simulink model "walkingRobot"  (R2019a)
settings: Solver=ode15s  StartTime=0.0  StopTime=10  EnableMultiTasking=on
InitFcn:
  | initAnglesR = evalSmoothTrajectory(curveData,0);
  | initAnglesL = evalSmoothTrajectory(curveData,-curveData.gaitPeriod/2);
values from neighbouring files (symbols this model uses):
  ankle_servo_kd = 8    [robotParameters.m]
  ankle_servo_ki = 4    [robotParameters.m]
  ankle_servo_kp = 20    [robotParameters.m]
  curveData = createSmoothTrajectory(ankle_motion,knee_motion,hip_motion,gaitPeriod)    [robotParameters.m]
  deriv_filter_coeff = 100    [robotParameters.m]
  foot_x = 8    [robotParameters.m]
  foot_y = 6    [robotParameters.m]
  foot_z = 1    [robotParameters.m]
  height_plane = 0.025    [robotParameters.m]
  hip_servo_kd = 20    [robotParameters.m]
  hip_servo_ki = 10    [robotParameters.m]
  hip_servo_kp = 60    [robotParameters.m]
  joint_stiffness = 1    [robotParameters.m]
  knee_servo_kd = 10    [robotParameters.m]
  knee_servo_ki = 5    [robotParameters.m]
  knee_servo_kp = 60    [robotParameters.m]
  lower_leg_length = 10    [robotParameters.m]
  N = 500    [plotSmoothTrajectory.m]
  plane_x = 25    [robotParameters.m]
  plane_y = 3    [robotParameters.m]
  torso_offset_x = -0.5    [robotParameters.m]
  torso_offset_z = -2    [robotParameters.m]
  torso_x = 5    [robotParameters.m]
  torso_y = 10    [robotParameters.m]
  torso_z = 8    [robotParameters.m]
  upper_leg_length = 10    [robotParameters.m]
undefined symbols (not defined in the file or in its folder): X, Y, Z
libraries: sm_lib x29, walkingRobotUtils x12, Contact_Forces_Lib x8, nesl_utility x4, simulink x1
settings Model: Creator=scastro  LastModifiedBy=scastro
settings DataIOCC: ReturnWorkspaceOutputs=off  OutputTimes=0:0.01:10
settings OptimizationCC: LifeSpan=inf
settings DebuggingCC: AllowSymbolicDim=off  SFUnexpectedBacktrackingDiag=warning  SFNoUnconditionalDefaultTransitionDiag=warning  SFExecutionAtInitializationDiag=none  UnitsInconsistencyMsg=none  ArithmeticOperatorsInVariantConditions=warning
settings SFSimCC: SimUseLocalCustomCode=off
settings RTWCC: RTWUseLocalCustomCode=off
settings CodeAppCC: StateflowObjectComments=on
settings GRTTargetCC: TargetLangStandard=C89/C90 (ANSI)  GeneratePreprocessorConditionals=Disable all
settings ConfigComp: CovMetricSettings=dw  CovHtmlReporting=on  CovSaveCumulativeToWorkspaceVar=on  CovSaveSingleToWorkspaceVar=on  CovExternalEMLEnable=off  CovSFcnEnable=off
settings SimscapeCC: SimscapeNormalizeSystem=off  SimscapeLogOpenViewer=on  SimscapeLogLimitData=off  SimscapeLogDataHistory=10000
settings ConfigurationSet: Description=SimMechanics 2G
settings DiagnosticsConfigSet: SimMechanicsRigidlyBoundBlock=none
settings ExplorerConfigSet: InternalSimMechanicsExplorerSettings="<ExplorerConfiguration><canonicalview>default</canonicalview><AnimationSetting><BasePlaybackSpeed>1.0</BasePlaybackSpeed><PlaybackSpeedFactor>1.0</PlaybackSpeedFactor></AnimationSetting><TilePanel><TileInfo><Tiles Columns=\"1\" Count=\"1\" Rows=\"1\"><Column Left=\"2\" Weight=\"1\"/><Column Left=\"1242\"/><Row Top=\"2\" Weight=\"1\"/><Row Top=\"924\"/><Tile Height=\"1\" Width=\"1\" X=\"0\" Y=\"0\"/></Tiles></TileInfo><SceneInfo><SceneViewer><BGColor><R>0.60000002384185791</R><G>0.60000002384185791</G><B>0.60000002384185791</B></BGColor><Camera><DoPerspective>off</DoPerspective><Position><X>3.5288544276265377</X><Y>-3.5929715781454834</Y><Z>1.702213827013187</Z></Position><Center><X>1.5263892499290903</X><Y>0.59161729631936055</Y><Z>-0.28619491412557885</Z></Center><Up><X>-0.24511053110164599</X><Y>0.31791313039198377</Y><Z>0.91588867722416945</Z></Up><ViewLimDist>1</ViewLimDist><YLim>1.3675114445300658</YLim><XLim>1.8438188260859925</XLim></Camera></SceneViewer></SceneInfo></TilePanel><MechEditorPanel><Cameras/><GfxPanelCameraMap/><VideoCreator><PlaybackSpeedRatio>1.0</PlaybackSpeedRatio><FrameRate>30</FrameRate><VideoFormat>Motion JPEG AVI</VideoFormat><FrameSize>auto</FrameSize></VideoCreator></MechEditorPanel></ExplorerConfiguration>"

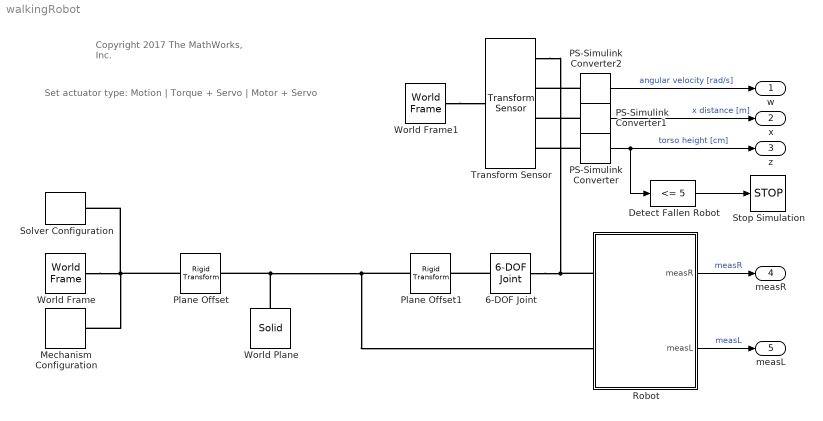
== system walkingRobot ==
  note: Set actuator type:
      | Motion | Torque + Servo | Motor + Servo
  note: Copyright 2017 The MathWorks, Inc.
  6-DOF Joint : sm_lib/Joints/6-DOF Joint  SenseConstraintForce=off  SenseConstraintForceX=off  SenseConstraintForceY=off  SenseConstraintForceZ=off  SenseConstraintTorque=off  SenseConstraintTorqueX=off  SenseConstraintTorqueY=off  SenseConstraintTorqueZ=off  SenseTotalForce=off  SenseTotalForceX=off  SenseTotalForceY=off  SenseTotalForceZ=off  SenseTotalTorque=off  SenseTotalTorqueX=off  SenseTotalTorqueY=off  SenseTotalTorqueZ=off  CompositeWrenchDir=FollowerOnBase  CompositeWrenchFrame=BaseFrame  PxEquilibriumPosition=0  PxEquilibriumPositionUnits=m  PxSpringStiffness=0  PxSpringStiffnessUnits=N/m  PxDampingCoefficient=world_damping  PxDampingCoefficientUnits=N/(m/s)  PxTorqueActuationMode=NoTorque  PxMotionActuationMode=ComputedMotion  PxSensePosition=off  PxSenseVelocity=off  PxSenseAcceleration=off  PxSenseTorqueForce=off  PxSenseLowerLimitTorqueForce=off  PxSenseUpperLimitTorqueForce=off  PxLowerLimitSpecify=off  PxLowerLimitBound=-1  PxLowerLimitBoundUnits=m  PxLowerLimitStiffness=1e6  PxLowerLimitStiffnessUnits=N/m  PxLowerLimitDamping=1e3  PxLowerLimitDampingUnits=N/(m/s)  PxLowerLimitTransitionRegionWidth=1e-4  PxLowerLimitTransitionRegionWidthUnits=m  PxUpperLimitSpecify=off  PxUpperLimitBound=1  PxUpperLimitBoundUnits=m  PxUpperLimitStiffness=1e6  PxUpperLimitStiffnessUnits=N/m  PxUpperLimitDamping=1e3  PxUpperLimitDampingUnits=N/(m/s)  PxUpperLimitTransitionRegionWidth=1e-4  PxUpperLimitTransitionRegionWidthUnits=m  PxPositionTargetSpecify=on  PxPositionTargetPriority=High  PxPositionTargetValue=0  PxPositionTargetValueUnits=m  PxVelocityTargetSpecify=off  PxVelocityTargetPriority=High  PxVelocityTargetValue=0  PxVelocityTargetValueUnits=m/s  PyEquilibriumPosition=0  PyEquilibriumPositionUnits=m  PySpringStiffness=0  PySpringStiffnessUnits=N/m  PyDampingCoefficient=world_damping  PyDampingCoefficientUnits=N/(m/s)  PyTorqueActuationMode=NoTorque  PyMotionActuationMode=ComputedMotion  PySensePosition=off  PySenseVelocity=off  PySenseAcceleration=off  PySenseTorqueForce=off  PySenseLowerLimitTorqueForce=off  PySenseUpperLimitTorqueForce=off  PyLowerLimitSpecify=off  PyLowerLimitBound=-1  PyLowerLimitBoundUnits=m  PyLowerLimitStiffness=1e6  PyLowerLimitStiffnessUnits=N/m  PyLowerLimitDamping=1e3  PyLowerLimitDampingUnits=N/(m/s)  PyLowerLimitTransitionRegionWidth=1e-4  PyLowerLimitTransitionRegionWidthUnits=m  PyUpperLimitSpecify=off  PyUpperLimitBound=1  PyUpperLimitBoundUnits=m  PyUpperLimitStiffness=1e6  PyUpperLimitStiffnessUnits=N/m  PyUpperLimitDamping=1e3  PyUpperLimitDampingUnits=N/(m/s)  PyUpperLimitTransitionRegionWidth=1e-4  PyUpperLimitTransitionRegionWidthUnits=m  PyPositionTargetSpecify=on  PyPositionTargetPriority=High  PyPositionTargetValue=0  PyPositionTargetValueUnits=m  PyVelocityTargetSpecify=off  PyVelocityTargetPriority=High  PyVelocityTargetValue=0  PyVelocityTargetValueUnits=m/s  PzEquilibriumPosition=0  PzEquilibriumPositionUnits=m  PzSpringStiffness=0  PzSpringStiffnessUnits=N/m  PzDampingCoefficient=world_damping  PzDampingCoefficientUnits=N/(m/s)  PzTorqueActuationMode=NoTorque  PzMotionActuationMode=ComputedMotion  PzSensePosition=off  PzSenseVelocity=off  PzSenseAcceleration=off  PzSenseTorqueForce=off  PzSenseLowerLimitTorqueForce=off  PzSenseUpperLimitTorqueForce=off  PzLowerLimitSpecify=off  PzLowerLimitBound=-1  PzLowerLimitBoundUnits=m  PzLowerLimitStiffness=1e6  PzLowerLimitStiffnessUnits=N/m  PzLowerLimitDamping=1e3  PzLowerLimitDampingUnits=N/(m/s)  PzLowerLimitTransitionRegionWidth=1e-4  PzLowerLimitTransitionRegionWidthUnits=m  PzUpperLimitSpecify=off  PzUpperLimitBound=1  PzUpperLimitBoundUnits=m  PzUpperLimitStiffness=1e6  PzUpperLimitStiffnessUnits=N/m  PzUpperLimitDamping=1e3  PzUpperLimitDampingUnits=N/(m/s)  PzUpperLimitTransitionRegionWidth=1e-4  PzUpperLimitTransitionRegionWidthUnits=m  PzPositionTargetSpecify=on  PzPositionTargetPriority=High  PzPositionTargetValue=init_height  PzPositionTargetValueUnits=cm  PzVelocityTargetSpecify=off  PzVelocityTargetPriority=High  PzVelocityTargetValue=0  PzVelocityTargetValueUnits=m/s  SphDefPosRotationMethod=None  SphDefPosRotationAngleUnits=deg  SphDefPosRotationStandardAxis=+Z  SphDefPosRotationAngle=0.0  SphDefPosRotationArbitraryAxis=[0 0 1]  SphDefPosFollAlignAxisA=+X  SphDefPosBaseAlignAxisA=+Y  SphDefPosFollAlignAxisB=+Y  SphDefPosBaseAlignAxisB=+Z  SphDefPosRotationSequenceAxes=FollowerAxes  SphDefPosRotationSequence=XYX  SphDefPosRotationSequenceAngles=[0 0 0]  SphDefPosRotationSequenceAnglesUnits=deg  SphDefPosRotationMatrix=[1 0 0; 0 1 0; 0 0 1]  SphEqPosRotationMethod=None  SphEqPosRotationAngleUnits=deg  SphEqPosRotationStandardAxis=+Z  SphEqPosRotationAngle=0.0  SphEqPosRotationArbitraryAxis=[0 0 1]  SphEqPosFollAlignAxisA=+X  SphEqPosBaseAlignAxisA=+Y  SphEqPosFollAlignAxisB=+Y  SphEqPosBaseAlignAxisB=+Z  SphEqPosRotationSequenceAxes=FollowerAxes  SphEqPosRotationSequence=XYX  SphEqPosRotationSequenceAngles=[0 0 0]  SphEqPosRotationSequenceAnglesUnits=deg  SphEqPosRotationMatrix=[1 0 0; 0 1 0; 0 0 1]  SphSpringStiffness=0  SphSpringStiffnessUnits=N*m/deg  SphDampingCoefficient=world_rot_damping  SphDampingCoefficientUnits=N*m/(rad/s)  SphActuateTorqueX=off  SphActuateTorqueY=off  SphActuateTorqueZ=off  SphActuateTorque=off  SphTorqueActuationMode=NoTorque  SphMotionActuationMode=ComputedMotion  SphActuationFrame=BaseFrame  SphSensePosition=off  SphSenseVelocityX=off  SphSenseVelocityY=off  SphSenseVelocityZ=off  SphSenseVelocity=off  SphSenseAccelerationX=off  SphSenseAccelerationY=off  SphSenseAccelerationZ=off  SphSenseAcceleration=off  SphSenseTorqueX=off  SphSenseTorqueY=off  SphSenseTorqueZ=off  SphSenseTorqueForce=off  SphSenseLowerLimitTorqueMag=off  SphSenseUpperLimitTorqueMag=off  SphSensingFrame=BaseFrame  SphLowerLimitSpecify=off  SphLowerLimitBound=15  SphLowerLimitBoundUnits=deg  SphLowerLimitStiffness=1e4  SphLowerLimitStiffnessUnits=N*m/deg  SphLowerLimitDamping=10  SphLowerLimitDampingUnits=N*m/(deg/s)  SphLowerLimitTransitionRegionWidth=0.1  SphLowerLimitTransitionRegionWidthUnits=deg  SphUpperLimitSpecify=off  SphUpperLimitBound=45  SphUpperLimitBoundUnits=deg  SphUpperLimitStiffness=1e4  SphUpperLimitStiffnessUnits=N*m/deg  SphUpperLimitDamping=10  SphUpperLimitDampingUnits=N*m/(deg/s)  SphUpperLimitTransitionRegionWidth=0.1  SphUpperLimitTransitionRegionWidthUnits=deg  SphPositionTargetRotationMethod=None  SphPositionTargetRotationAngleUnits=deg  SphPositionTargetRotationStandardAxis=+Z  SphPositionTargetRotationAngle=0.0  SphPositionTargetRotationArbitraryAxis=[0 0 1]  SphPositionTargetFollAlignAxisA=+X  SphPositionTargetBaseAlignAxisA=+Y  SphPositionTargetFollAlignAxisB=+Y  SphPositionTargetBaseAlignAxisB=+Z  SphPositionTargetRotationSequenceAxes=FollowerAxes  SphPositionTargetRotationSequence=XYX  SphPositionTargetRotationSequenceAngles=[0 0 0]  SphPositionTargetRotationSequenceAnglesUnits=deg  SphPositionTargetRotationMatrix=eye(3)  SphPositionTargetSpecify=off  SphPositionTargetPriority=High  SphVelocityTargetValue=[0 0 0]  SphVelocityTargetValueUnits=deg/s  SphVelocityTargetSpecify=off  SphVelocityTargetPriority=High  SphVelocityTargetInFollowerFrame=on
  Detect Fallen Robot : simulink/Logic and Bit Operations/Compare To Constant  relop=<=  const=5  OutDataTypeStr=boolean
  Mechanism Configuration : sm_lib/Utilities/Mechanism Configuration  UniformGravity=Constant  GravityVector=[0 0 -9.80665]  GravityUnits=m/s^2  LinearizationDelta=0.001
  PS-Simulink Converter : nesl_utility/PS-Simulink Converter  PhysicalDomain=network_engine_domain  SubClassName=ps_output  LeftPortType=input  RightPortType=output  PseudoPeriodic=off  Frequencies=[]  Unit=cm  AffineConversion=off
  PS-Simulink Converter1 : nesl_utility/PS-Simulink Converter  PhysicalDomain=network_engine_domain  SubClassName=ps_output  LeftPortType=input  RightPortType=output  PseudoPeriodic=off  Frequencies=[]  Unit=m  AffineConversion=off
  PS-Simulink Converter2 : nesl_utility/PS-Simulink Converter  PhysicalDomain=network_engine_domain  SubClassName=ps_output  LeftPortType=input  RightPortType=output  PseudoPeriodic=off  Frequencies=[]  Unit=rad/s  AffineConversion=off
  Plane Offset : sm_lib/Frames and Transforms/Rigid Transform  TranslationMethod=StandardAxis  TranslationStandardOffset=height_plane/2  TranslationLengthUnit=m  TranslationStandardAxis=-Z  TranslationCartesianOffset=[0 0 0]  TranslationROffset=0  TranslationROffsetUnits=m  TranslationZOffset=0  TranslationZOffsetUnits=m  TranslationThetaOffset=0  TranslationThetaOffsetUnits=deg  RotationMethod=None  RotationAngleUnits=deg  RotationStandardAxis=+Z  RotationAngle=0.0  RotationArbitraryAxis=[0 0 1]  FollAlignAxisA=+X  BaseAlignAxisA=+Y  FollAlignAxisB=+Y  BaseAlignAxisB=+Z  RotationSequenceAxes=FollowerAxes  RotationSequence=XYX  RotationSequenceAngles=[0 0 0]  RotationSequenceAnglesUnits=deg  RotationMatrix=[1 0 0; 0 1 0; 0 0 1]
  Plane Offset1 : sm_lib/Frames and Transforms/Rigid Transform  TranslationMethod=StandardAxis  TranslationStandardOffset=height_plane/2  TranslationLengthUnit=m  TranslationStandardAxis=+Z  TranslationCartesianOffset=[0 0 0]  TranslationROffset=0  TranslationROffsetUnits=m  TranslationZOffset=0  TranslationZOffsetUnits=m  TranslationThetaOffset=0  TranslationThetaOffsetUnits=deg  RotationMethod=None  RotationAngleUnits=deg  RotationStandardAxis=+Z  RotationAngle=0.0  RotationArbitraryAxis=[0 0 1]  FollAlignAxisA=+X  BaseAlignAxisA=+Y  FollAlignAxisB=+Y  BaseAlignAxisB=+Z  RotationSequenceAxes=FollowerAxes  RotationSequence=XYX  RotationSequenceAngles=[0 0 0]  RotationSequenceAnglesUnits=deg  RotationMatrix=[1 0 0; 0 1 0; 0 0 1]
  Robot : Subsystem
  Solver Configuration : nesl_utility/Solver Configuration  PhysicalDomain=network_engine_domain  SubClassName=solver  LeftPortType=input  RightPortType=generic  Tones=[]  Harmonics=[]  SimulateNoise=off  Profile=off  UseLocalSampling=off  EnableSwitchedLinearOptims=on  FrequencyDomain=off  UseCCode=off  RelTol=0.001  AbsTol=1e-06  MinStep=1e-09  ToWorkspace=off  RevertToSquareIcSolve=off  NumHomotopyIterations=100  PhasorMode=off  PhasorModeNumHarmonics=1  DoDC=off  ResidualTolerance=1e-09  UseLocalSolver=off  LocalSolverChoice=NE_TRAPEZOIDAL_ADVANCER  LocalSolverSampleTime=0.001  DoFixedCost=off  MaxNonlinIter=3  MaxModeIter=2  LinearAlgebra=Sparse  EquationFormulation=NE_TIME_EF  DelaysMemoryBudget=1024  AutomaticFiltering=on  FilteringTimeConstant=0.001  PartitionStorageMethod=AS_NEEDED  PartitionMemoryBudget=1024  PartitionMethod=FAST
  Stop Simulation : Stop
  Transform Sensor : sm_lib/Frames and Transforms/Transform Sensor  MeasurementFrame=World  SenseAngle=off  SenseAxis=off  SenseAngle1=off  SenseAngle2=off  SenseAngle3=off  SenseQ=off  SenseR=off  SenseOmegaX=off  SenseOmegaY=off  SenseOmegaZ=on  SenseOmega1=off  SenseOmega2=off  SenseOmega3=off  SenseQDot=off  SenseRDot=off  SenseAlphaX=off  SenseAlphaY=off  SenseAlphaZ=off  SenseAlpha1=off  SenseAlpha2=off  SenseAlpha3=off  SenseQDDot=off  SenseRDDot=off  SenseX=on  SenseY=off  SenseZ=on  SenseRad=off  SenseAzim=off  SenseDist=off  SenseInc=off  SenseXDot=off  SenseYDot=off  SenseZDot=off  SenseRadDot=off  SenseAzimDot=off  SenseDistDot=off  SenseIncDot=off  SenseXDDot=off  SenseYDDot=off  SenseZDDot=off  SenseRadDDot=off  SenseAzimDDot=off  SenseDistDDot=off  SenseIncDDot=off
  World Frame : sm_lib/Frames and Transforms/World Frame
  World Frame1 : sm_lib/Frames and Transforms/World Frame
  World Plane : sm_lib/Body Elements/Solid  InertiaType=CalculateFromGeometry  Mass=1  MassUnits=kg  CenterOfMass=[0 0 0]  CenterOfMassUnits=m  MomentsOfInertia=[1 1 1]  MomentsOfInertiaUnits=kg*m^2  ProductsOfInertia=[0 0 0]  ProductsOfInertiaUnits=kg*m^2  BasedOnType=Density  Density=density  DensityUnits=kg/(m^3)  DoExposeReferenceFrame=on  SerializedFrames=<Frames/>  GraphicType=FromGeometry  MarkerShape=Sphere  MarkerSize=10  MarkerSizeUnits=m  GraphicVisPropType=SimpleVisualProperties  GraphicDiffuseColor=[1.0 1.0 0.8]  GraphicSpecularColor=[0.5 0.5 0.5 1.0]  GraphicAmbientColor=[0.15 0.15 0.15 1.0]  GraphicEmissiveColor=[0.0 0.0 0.0 1.0]  GraphicShininess=75  GraphicOpacity=0.5  GeometryShape=Brick  RectangleSize=[1 1]  RectangleSizeUnits=m  BrickDimensions="[plane_x plane_y  height_plane]"  BrickDimensionUnits=m  CylinderRadius=1  CylinderRadiusUnits=m  CylinderLength=1  CylinderLengthUnits=m  SphereRadius=1  SphereRadiusUnits=m  EllipsoidRadii=[1 1 1]  EllipsoidRadiiUnits=m  ExtrusionCrossSection=[1 1; -1 1; -1 -1; 1 -1]  ExtrusionCrossSectionUnits=m  ExtrusionLength=1  ExtrusionLengthUnits=m  PolygonNumSides=3  PolygonOuterRadius=1  PolygonOuterRadiusUnits=m  ExtGeomFileType=STL  ExtGeomFileUnits=m  RevolutionCrossSection=[1 1; 1 -1; 2 -1; 2 1]  RevolutionCrossSectionUnits=m  RevolutionExtent=Full  RevolutionAngle=180  RevolutionAngleUnits=deg
  w : Outport
  x : Outport  Port=2
  z : Outport  Port=3
  measR : Outport  Port=4
  measL : Outport  Port=5
  wires:
  PS-Simulink Converter/1 -> z/1, Detect Fallen Robot/1  "torso height [cm]"
  PS-Simulink Converter1/1 -> x/1  "x distance [m]"
  Detect Fallen Robot/1 -> Stop Simulation/1
  PS-Simulink Converter2/1 -> w/1  "angular velocity [rad/s]"
  Robot/1(measR) -> measR/1  "measR"
  Robot/2(measL) -> measL/1  "measL"
  connections:
  World Frame1/RConn1 -- Transform Sensor/LConn1
  PS-Simulink Converter/LConn1 -- Transform Sensor/RConn4
  PS-Simulink Converter1/LConn1 -- Transform Sensor/RConn3
  PS-Simulink Converter2/LConn1 -- Transform Sensor/RConn2
  Plane Offset/LConn1 -- World Frame/RConn1 -- Mechanism Configuration/RConn1 -- Solver Configuration/RConn1
  World Plane/RConn1 -- Plane Offset/RConn1 -- Plane Offset1/LConn1 -- Robot/LConn2
  6-DOF Joint/LConn1 -- Plane Offset1/RConn1
  Transform Sensor/RConn1 -- 6-DOF Joint/RConn1 -- Robot/LConn1

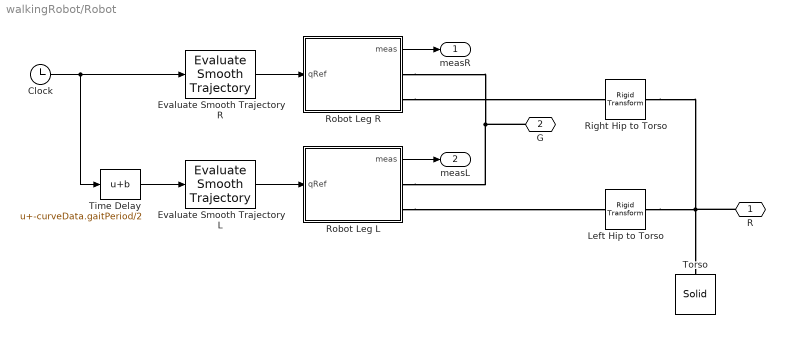
== system walkingRobot/Robot ==
  Clock : Clock
  Evaluate Smooth Trajectory L : walkingRobotUtils/Evaluate Smooth  Trajectory  SystemSampleTime=-1
  Evaluate Smooth Trajectory R : walkingRobotUtils/Evaluate Smooth  Trajectory  SystemSampleTime=-1
  Left Hip to Torso : sm_lib/Frames and Transforms/Rigid Transform  TranslationMethod=Cartesian  TranslationStandardOffset=0  TranslationLengthUnit=cm  TranslationStandardAxis=+Z  TranslationCartesianOffset=[torso_offset_x torso_y/2 torso_offset_z]  TranslationROffset=0  TranslationROffsetUnits=m  TranslationZOffset=0  TranslationZOffsetUnits=m  TranslationThetaOffset=0  TranslationThetaOffsetUnits=deg  RotationMethod=None  RotationAngleUnits=deg  RotationStandardAxis=+Z  RotationAngle=0.0  RotationArbitraryAxis=[0 0 1]  FollAlignAxisA=+X  BaseAlignAxisA=+Y  FollAlignAxisB=+Y  BaseAlignAxisB=+Z  RotationSequenceAxes=FollowerAxes  RotationSequence=XYX  RotationSequenceAngles=[0 0 0]  RotationSequenceAnglesUnits=deg  RotationMatrix=[1 0 0; 0 1 0; 0 0 1]
  Right Hip to Torso : sm_lib/Frames and Transforms/Rigid Transform  TranslationMethod=Cartesian  TranslationStandardOffset=0  TranslationLengthUnit=cm  TranslationStandardAxis=+Z  TranslationCartesianOffset=[torso_offset_x -torso_y/2 torso_offset_z]  TranslationROffset=0  TranslationROffsetUnits=m  TranslationZOffset=0  TranslationZOffsetUnits=m  TranslationThetaOffset=0  TranslationThetaOffsetUnits=deg  RotationMethod=None  RotationAngleUnits=deg  RotationStandardAxis=+Z  RotationAngle=0.0  RotationArbitraryAxis=[0 0 1]  FollAlignAxisA=+X  BaseAlignAxisA=+Y  FollAlignAxisB=+Y  BaseAlignAxisB=+Z  RotationSequenceAxes=FollowerAxes  RotationSequence=XYX  RotationSequenceAngles=[0 0 0]  RotationSequenceAnglesUnits=deg  RotationMatrix=[1 0 0; 0 1 0; 0 0 1]
  Robot Leg L : Subsystem
  Robot Leg R : Subsystem
  Time Delay : Bias  Bias=-curveData.gaitPeriod/2
  Torso : sm_lib/Body Elements/Solid  InertiaType=CalculateFromGeometry  Mass=1  MassUnits=kg  CenterOfMass=[0 0 0]  CenterOfMassUnits=m  MomentsOfInertia=[1 1 1]  MomentsOfInertiaUnits=kg*m^2  ProductsOfInertia=[1 1 1]  ProductsOfInertiaUnits=kg*m^2  BasedOnType=Density  Density=density  DensityUnits=kg/m^3  DoExposeReferenceFrame=on  SerializedFrames=<Frames/>  GraphicType=FromGeometry  MarkerShape=Sphere  MarkerSize=10  GraphicVisPropType=SimpleVisualProperties  GraphicDiffuseColor=[0.5 0.5 0.5]  GraphicSpecularColor=[0.5 0.5 0.5 1.0]  GraphicAmbientColor=[0.15 0.15 0.15 1.0]  GraphicEmissiveColor=[0.0 0.0 0.0 1.0]  GraphicShininess=75  GraphicOpacity=1.0  GeometryShape=Brick  RectangleSize=[1 1]  RectangleSizeUnits=m  BrickDimensions=[torso_x torso_y torso_z]  BrickDimensionUnits=cm  CylinderRadius=1  CylinderRadiusUnits=m  CylinderLength=1  CylinderLengthUnits=m  SphereRadius=1  SphereRadiusUnits=m  EllipsoidRadii=[1 1 1]  EllipsoidRadiiUnits=m  ExtrusionCrossSection=[1 1; -1 1; -1 -1; 1 -1]  ExtrusionCrossSectionUnits=m  ExtrusionLength=1  ExtrusionLengthUnits=m  PolygonNumSides=3  PolygonOuterRadius=1  PolygonOuterRadiusUnits=m  ExtGeomFileType=STEP  ExtGeomFileUnits=m  RevolutionCrossSection=[1 1; 1 -1; 2 -1; 2 1]  RevolutionCrossSectionUnits=m  RevolutionExtent=Full  RevolutionAngle=180  RevolutionAngleUnits=deg
  R : PMIOPort  Side=Left
  G : PMIOPort  Port=2  Side=Left
  measR : Outport
  measL : Outport  Port=2
  wires:
  Robot Leg L/1(meas) -> measL/1
  Robot Leg R/1(meas) -> measR/1
  Clock/1 -> Evaluate Smooth Trajectory R/1, Time Delay/1
  Evaluate Smooth Trajectory R/1 -> Robot Leg R/1(qRef)
  Time Delay/1 -> Evaluate Smooth Trajectory L/1
  Evaluate Smooth Trajectory L/1 -> Robot Leg L/1(qRef)
  connections:
  Robot Leg R/RConn2 -- Right Hip to Torso/RConn1
  Robot Leg L/RConn2 -- Left Hip to Torso/RConn1
  Right Hip to Torso/LConn1 -- Torso/RConn1 -- R/RConn1 -- Left Hip to Torso/LConn1
  Robot Leg R/RConn1 -- Robot Leg L/RConn1 -- G/RConn1

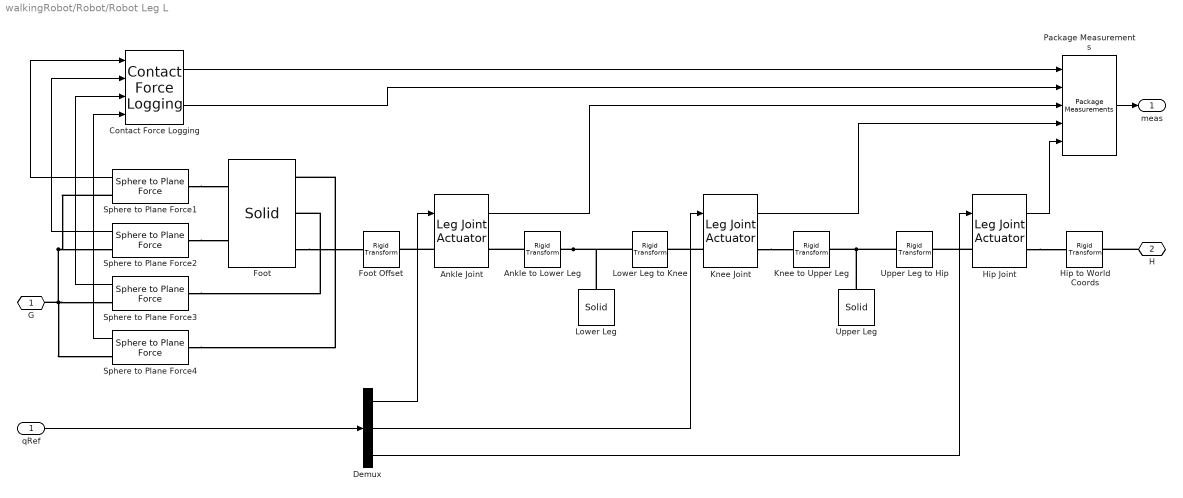
== system walkingRobot/Robot/Robot Leg L ==
  qRef : Inport
  Ankle Joint : walkingRobotUtils/Leg Joint Actuator  k=joint_stiffness  d=joint_damping  initAngle=initAnglesL(1)  Tf=motion_time_constant  Kp=ankle_servo_kp  Ki=ankle_servo_ki  Kd=ankle_servo_kd  N=deriv_filter_coeff  Tmax=max_torque
  Ankle to Lower Leg : sm_lib/Frames and Transforms/Rigid Transform  TranslationMethod=Cartesian  TranslationStandardOffset=0  TranslationLengthUnit=cm  TranslationStandardAxis=+Z  TranslationCartesianOffset=[0 lower_leg_length/2 0]  TranslationROffset=0  TranslationROffsetUnits=m  TranslationZOffset=0  TranslationZOffsetUnits=m  TranslationThetaOffset=0  TranslationThetaOffsetUnits=deg  RotationMethod=StandardAxis  RotationAngleUnits=deg  RotationStandardAxis=+X  RotationAngle=-90  RotationArbitraryAxis=[0 0 1]  FollAlignAxisA=+X  BaseAlignAxisA=+Y  FollAlignAxisB=+Y  BaseAlignAxisB=+Z  RotationSequenceAxes=FollowerAxes  RotationSequence=XYX  RotationSequenceAngles=[0 0 0]  RotationSequenceAnglesUnits=deg  RotationMatrix=[1 0 0; 0 1 0; 0 0 1]
  Contact Force Logging : walkingRobotUtils/Contact Force Logging  SystemSampleTime=-1
  Demux : Demux  Outputs=3
  Foot : sm_lib/Body Elements/Solid  InertiaType=CalculateFromGeometry  Mass=1  MassUnits=kg  CenterOfMass=[0 0 0]  CenterOfMassUnits=m  MomentsOfInertia=[1 1 1]  MomentsOfInertiaUnits=kg*m^2  ProductsOfInertia=[0 0 0]  ProductsOfInertiaUnits=kg*m^2  BasedOnType=Density  Density=foot_density  DensityUnits=kg/(m^3)  DoExposeReferenceFrame=off  SerializedFrames=<Frames><Frame><Id>Frame1</Id><Value><Name>F1</Name><Origin><Source>GeometricFeature</Source><FeatureName>+x -y -z point</FeatureName></Origin><PrimaryAxis><DefinedDirection>+Z</DefinedDirection><Source>ReferenceFrame</Source><SourceDirection>+Z</SourceDirection><FeatureName></FeatureName></PrimaryAxis><SecondaryAxis><DefinedDirection>+X</DefinedDirection><Source>ReferenceFrame</Source><SourceDirection>+X</SourceDirection><FeatureName></FeatureName></SecondaryAxis></Value></Frame><Frame><Id>Frame2</Id><Value><Name>F2</Name><Origin><Source>GeometricFeature</Source><FeatureName>+x +y -z point</FeatureName></Origin><PrimaryAxis><DefinedDirection>+Z</DefinedDirection><Source>ReferenceFrame</Source><SourceDirection>+Z</SourceDirection><FeatureName></FeatureName></PrimaryAxis><SecondaryAxis><DefinedDirection>+X</DefinedDirection><Source>ReferenceFrame</Source><SourceDirection>+X</SourceDirection><FeatureName></FeatureName></SecondaryAxis></Value></Frame><Frame><Id>Frame3</Id><Value><Name>F3</Name><Origin><Source>GeometricFeature</Source><FeatureName>-x -y -z point</FeatureName></Origin><PrimaryAxis><DefinedDirection>+Z</DefinedDirection><Source>ReferenceFrame</Source><SourceDirection>+Z</SourceDirection><FeatureName></FeatureName></PrimaryAxis><SecondaryAxis><DefinedDirection>+X</DefinedDirection><Source>ReferenceFrame</Source><SourceDirection>+X</SourceDirection><FeatureName></FeatureName></SecondaryAxis></Value></Frame><Frame><Id>Frame4</Id><Value><Name>F4</Name><Origin><Source>GeometricFeature</Source><FeatureName>-x +y -z point</FeatureName></Origin><PrimaryAxis><DefinedDirection>+Z</DefinedDirection><Source>ReferenceFrame</Source><SourceDirection>+Z</SourceDirection><FeatureName></FeatureName></PrimaryAxis><SecondaryAxis><DefinedDirection>+X</DefinedDirection><Source>ReferenceFrame</Source><SourceDirection>+X</SourceDirection><FeatureName></FeatureName></SecondaryAxis></Value></Frame><Frame><Id>Frame5</Id><Value><Name>A</Name><Origin><Source>GeometricFeature</Source><FeatureName>+z surface</FeatureName></Origin><PrimaryAxis><DefinedDirection>+Z</DefinedDirection><Source>ReferenceFrame</Source><SourceDirection>-Y</SourceDirection><FeatureName></FeatureName></PrimaryAxis><SecondaryAxis><DefinedDirection>+X</DefinedDirection><Source>ReferenceFrame</Source><SourceDirection>+X</SourceDirection><FeatureName></FeatureName></SecondaryAxis></Value></Frame></Frames>  GraphicType=FromGeometry  MarkerShape=Sphere  MarkerSize=10  MarkerSizeUnits=m  GraphicVisPropType=SimpleVisualProperties  GraphicDiffuseColor=[0.5 0.5 0.5]  GraphicSpecularColor=[0.5 0.5 0.5 1.0]  GraphicAmbientColor=[0.15 0.15 0.15 1.0]  GraphicEmissiveColor=[0.0 0.0 0.0 1.0]  GraphicShininess=75  GraphicOpacity=1.0  GeometryShape=Brick  RectangleSize=[1 1]  RectangleSizeUnits=m  BrickDimensions=[foot_x foot_y foot_z]  BrickDimensionUnits=cm  CylinderRadius=1  CylinderRadiusUnits=m  CylinderLength=1  CylinderLengthUnits=m  SphereRadius=1  SphereRadiusUnits=m  EllipsoidRadii=[1 1 1]  EllipsoidRadiiUnits=m  ExtrusionCrossSection=[1 1; -1 1; -1 -1; 1 -1]  ExtrusionCrossSectionUnits=m  ExtrusionLength=1  ExtrusionLengthUnits=m  PolygonNumSides=3  PolygonOuterRadius=1  PolygonOuterRadiusUnits=m  ExtGeomFileType=STL  ExtGeomFileUnits=m  RevolutionCrossSection=[1 1; 1 -1; 2 -1; 2 1]  RevolutionCrossSectionUnits=m  RevolutionExtent=Full  RevolutionAngle=180  RevolutionAngleUnits=deg
  Foot Offset : sm_lib/Frames and Transforms/Rigid Transform  TranslationMethod=Cartesian  TranslationStandardOffset=0  TranslationLengthUnit=cm  TranslationStandardAxis=+Z  TranslationCartesianOffset=foot_offset  TranslationROffset=0  TranslationROffsetUnits=m  TranslationZOffset=0  TranslationZOffsetUnits=m  TranslationThetaOffset=0  TranslationThetaOffsetUnits=deg  RotationMethod=None  RotationAngleUnits=deg  RotationStandardAxis=+X  RotationAngle=-90  RotationArbitraryAxis=[0 0 1]  FollAlignAxisA=+X  BaseAlignAxisA=+Y  FollAlignAxisB=+Y  BaseAlignAxisB=+Z  RotationSequenceAxes=FollowerAxes  RotationSequence=XYX  RotationSequenceAngles=[0 0 0]  RotationSequenceAnglesUnits=deg  RotationMatrix=[1 0 0; 0 1 0; 0 0 1]
  Hip Joint : walkingRobotUtils/Leg Joint Actuator  k=joint_stiffness  d=joint_damping  initAngle=initAnglesL(3)  Tf=motion_time_constant  Kp=hip_servo_kp  Ki=hip_servo_ki  Kd=hip_servo_kd  N=deriv_filter_coeff  Tmax=max_torque
  Hip to World Coords : sm_lib/Frames and Transforms/Rigid Transform  TranslationMethod=None  TranslationStandardOffset=0  TranslationLengthUnit=cm  TranslationStandardAxis=+Z  TranslationCartesianOffset=[0 0 upper_leg_length/2]  TranslationROffset=0  TranslationROffsetUnits=m  TranslationZOffset=0  TranslationZOffsetUnits=m  TranslationThetaOffset=0  TranslationThetaOffsetUnits=deg  RotationMethod=StandardAxis  RotationAngleUnits=deg  RotationStandardAxis=+X  RotationAngle=-90  RotationArbitraryAxis=[0 0 1]  FollAlignAxisA=+X  BaseAlignAxisA=+Y  FollAlignAxisB=+Y  BaseAlignAxisB=+Z  RotationSequenceAxes=FollowerAxes  RotationSequence=XYX  RotationSequenceAngles=[0 0 0]  RotationSequenceAnglesUnits=deg  RotationMatrix=[1 0 0; 0 1 0; 0 0 1]
  Knee Joint : walkingRobotUtils/Leg Joint Actuator  k=joint_stiffness  d=joint_damping  initAngle=initAnglesL(2)  Tf=motion_time_constant  Kp=knee_servo_kp  Ki=knee_servo_ki  Kd=knee_servo_kd  N=deriv_filter_coeff  Tmax=max_torque
  Knee to Upper Leg : sm_lib/Frames and Transforms/Rigid Transform  TranslationMethod=Cartesian  TranslationStandardOffset=0  TranslationLengthUnit=cm  TranslationStandardAxis=+Z  TranslationCartesianOffset=[0 upper_leg_length/2 0]  TranslationROffset=0  TranslationROffsetUnits=m  TranslationZOffset=0  TranslationZOffsetUnits=m  TranslationThetaOffset=0  TranslationThetaOffsetUnits=deg  RotationMethod=StandardAxis  RotationAngleUnits=deg  RotationStandardAxis=+X  RotationAngle=-90  RotationArbitraryAxis=[0 0 1]  FollAlignAxisA=+X  BaseAlignAxisA=+Y  FollAlignAxisB=+Y  BaseAlignAxisB=+Z  RotationSequenceAxes=FollowerAxes  RotationSequence=XYX  RotationSequenceAngles=[0 0 0]  RotationSequenceAnglesUnits=deg  RotationMatrix=[1 0 0; 0 1 0; 0 0 1]
  Lower Leg : sm_lib/Body Elements/Solid  InertiaType=CalculateFromGeometry  Mass=1  MassUnits=kg  CenterOfMass=[0 0 0]  CenterOfMassUnits=m  MomentsOfInertia=[1 1 1]  MomentsOfInertiaUnits=kg*m^2  ProductsOfInertia=[1 1 1]  ProductsOfInertiaUnits=kg*m^2  BasedOnType=Density  Density=density  DensityUnits=kg/m^3  DoExposeReferenceFrame=on  SerializedFrames=<Frames/>  GraphicType=FromGeometry  MarkerShape=Sphere  MarkerSize=10  GraphicVisPropType=SimpleVisualProperties  GraphicDiffuseColor=[0.4 0.4 1.0]  GraphicSpecularColor=[0.5 0.5 0.5 1.0]  GraphicAmbientColor=[0.15 0.15 0.15 1.0]  GraphicEmissiveColor=[0.0 0.0 0.0 1.0]  GraphicShininess=75  GraphicOpacity=1.0  GeometryShape=Cylinder  RectangleSize=[1 1]  RectangleSizeUnits=m  BrickDimensions=[1 1 1]  BrickDimensionUnits=m  CylinderRadius=leg_radius  CylinderRadiusUnits=cm  CylinderLength=lower_leg_length  CylinderLengthUnits=cm  SphereRadius=1  SphereRadiusUnits=m  EllipsoidRadii=[1 1 1]  EllipsoidRadiiUnits=m  ExtrusionCrossSection=[1 1; -1 1; -1 -1; 1 -1]  ExtrusionCrossSectionUnits=m  ExtrusionLength=1  ExtrusionLengthUnits=m  PolygonNumSides=3  PolygonOuterRadius=1  PolygonOuterRadiusUnits=m  ExtGeomFileType=STEP  ExtGeomFileUnits=m  RevolutionCrossSection=[1 1; 1 -1; 2 -1; 2 1]  RevolutionCrossSectionUnits=m  RevolutionExtent=Full  RevolutionAngle=180  RevolutionAngleUnits=deg
  Lower Leg to Knee : sm_lib/Frames and Transforms/Rigid Transform  TranslationMethod=Cartesian  TranslationStandardOffset=0  TranslationLengthUnit=cm  TranslationStandardAxis=+Z  TranslationCartesianOffset=[0 0 lower_leg_length/2]  TranslationROffset=0  TranslationROffsetUnits=m  TranslationZOffset=0  TranslationZOffsetUnits=m  TranslationThetaOffset=0  TranslationThetaOffsetUnits=deg  RotationMethod=StandardAxis  RotationAngleUnits=deg  RotationStandardAxis=+X  RotationAngle=90  RotationArbitraryAxis=[0 0 1]  FollAlignAxisA=+X  BaseAlignAxisA=+Y  FollAlignAxisB=+Y  BaseAlignAxisB=+Z  RotationSequenceAxes=FollowerAxes  RotationSequence=XYX  RotationSequenceAngles=[0 0 0]  RotationSequenceAnglesUnits=deg  RotationMatrix=[1 0 0; 0 1 0; 0 0 1]
  Package Measurements : walkingRobotUtils/Package  Measurements  SystemSampleTime=-1
  Sphere to Plane Force{1..4} (4 alike) : Contact_Forces_Lib/3D/Sphere to Plane Force  sphere_rad=contact_point_radius  plane_lenx=plane_x  plane_leny=plane_y  plane_depth=height_plane/2  force_law=Linear  k_contact=contact_stiffness  b_contact=contact_damping  pen_full_damp_F=1e-4  pen_exponent=1  custom_param_1=1  custom_param_2=1  friction_law=Stick-Slip Continuous  mu_kinetic=mu_k  mu_static=mu_s  v_thr=mu_vth  vis_on=off  vis_opc_en=0  vis_len_plaBz=0.005  vis_clr=[0.9 0.2 0.2]  vis_opc=0.7
  Upper Leg : sm_lib/Body Elements/Solid  InertiaType=CalculateFromGeometry  Mass=1  MassUnits=kg  CenterOfMass=[0 0 0]  CenterOfMassUnits=m  MomentsOfInertia=[1 1 1]  MomentsOfInertiaUnits=kg*m^2  ProductsOfInertia=[1 1 1]  ProductsOfInertiaUnits=kg*m^2  BasedOnType=Density  Density=density  DensityUnits=kg/m^3  DoExposeReferenceFrame=on  SerializedFrames=<Frames/>  GraphicType=FromGeometry  MarkerShape=Sphere  MarkerSize=10  GraphicVisPropType=SimpleVisualProperties  GraphicDiffuseColor=[1.0 0.4 0.4]  GraphicSpecularColor=[0.5 0.5 0.5 1.0]  GraphicAmbientColor=[0.15 0.15 0.15 1.0]  GraphicEmissiveColor=[0.0 0.0 0.0 1.0]  GraphicShininess=75  GraphicOpacity=1.0  GeometryShape=Cylinder  RectangleSize=[1 1]  RectangleSizeUnits=m  BrickDimensions=[1 1 1]  BrickDimensionUnits=m  CylinderRadius=leg_radius  CylinderRadiusUnits=cm  CylinderLength=upper_leg_length  CylinderLengthUnits=cm  SphereRadius=1  SphereRadiusUnits=m  EllipsoidRadii=[1 1 1]  EllipsoidRadiiUnits=m  ExtrusionCrossSection=[1 1; -1 1; -1 -1; 1 -1]  ExtrusionCrossSectionUnits=m  ExtrusionLength=1  ExtrusionLengthUnits=m  PolygonNumSides=3  PolygonOuterRadius=1  PolygonOuterRadiusUnits=m  ExtGeomFileType=STEP  ExtGeomFileUnits=m  RevolutionCrossSection=[1 1; 1 -1; 2 -1; 2 1]  RevolutionCrossSectionUnits=m  RevolutionExtent=Full  RevolutionAngle=180  RevolutionAngleUnits=deg
  Upper Leg to Hip : sm_lib/Frames and Transforms/Rigid Transform  TranslationMethod=Cartesian  TranslationStandardOffset=0  TranslationLengthUnit=cm  TranslationStandardAxis=+Z  TranslationCartesianOffset=[0 0 upper_leg_length/2]  TranslationROffset=0  TranslationROffsetUnits=m  TranslationZOffset=0  TranslationZOffsetUnits=m  TranslationThetaOffset=0  TranslationThetaOffsetUnits=deg  RotationMethod=StandardAxis  RotationAngleUnits=deg  RotationStandardAxis=+X  RotationAngle=90  RotationArbitraryAxis=[0 0 1]  FollAlignAxisA=+X  BaseAlignAxisA=+Y  FollAlignAxisB=+Y  BaseAlignAxisB=+Z  RotationSequenceAxes=FollowerAxes  RotationSequence=XYX  RotationSequenceAngles=[0 0 0]  RotationSequenceAnglesUnits=deg  RotationMatrix=[1 0 0; 0 1 0; 0 0 1]
  G : PMIOPort  Side=Right
  H : PMIOPort  Port=2  Side=Right
  meas : Outport
  wires:
  Demux/1 -> Ankle Joint/1
  Demux/2 -> Knee Joint/1
  Demux/3 -> Hip Joint/1
  Package Measurements/1 -> meas/1
  Hip Joint/1 -> Package Measurements/5
  Knee Joint/1 -> Package Measurements/4
  Ankle Joint/1 -> Package Measurements/3
  Sphere to Plane Force1/1 -> Contact Force Logging/1
  Sphere to Plane Force2/1 -> Contact Force Logging/2
  Sphere to Plane Force3/1 -> Contact Force Logging/3
  Sphere to Plane Force4/1 -> Contact Force Logging/4
  qRef/1 -> Demux/1
  Contact Force Logging/1 -> Package Measurements/1
  Contact Force Logging/2 -> Package Measurements/2
  connections:
  G/RConn1 -- Sphere to Plane Force4/RConn1 -- Sphere to Plane Force3/RConn1 -- Sphere to Plane Force1/RConn1 -- Sphere to Plane Force2/RConn1
  Knee Joint/RConn1 -- Knee to Upper Leg/LConn1
  Ankle to Lower Leg/LConn1 -- Ankle Joint/RConn1
  Sphere to Plane Force2/LConn1 -- Foot/RConn2
  Sphere to Plane Force1/LConn1 -- Foot/RConn1
  Sphere to Plane Force4/LConn1 -- Foot/LConn1
  Sphere to Plane Force3/LConn1 -- Foot/LConn2
  Ankle to Lower Leg/RConn1 -- Lower Leg/RConn1 -- Lower Leg to Knee/LConn1
  Ankle Joint/LConn1 -- Foot Offset/RConn1
  Upper Leg to Hip/LConn1 -- Upper Leg/RConn1 -- Knee to Upper Leg/RConn1
  Hip Joint/LConn1 -- Upper Leg to Hip/RConn1
  Knee Joint/LConn1 -- Lower Leg to Knee/RConn1
  H/RConn1 -- Hip to World Coords/RConn1
  Hip Joint/RConn1 -- Hip to World Coords/LConn1
  Foot/LConn3 -- Foot Offset/LConn1

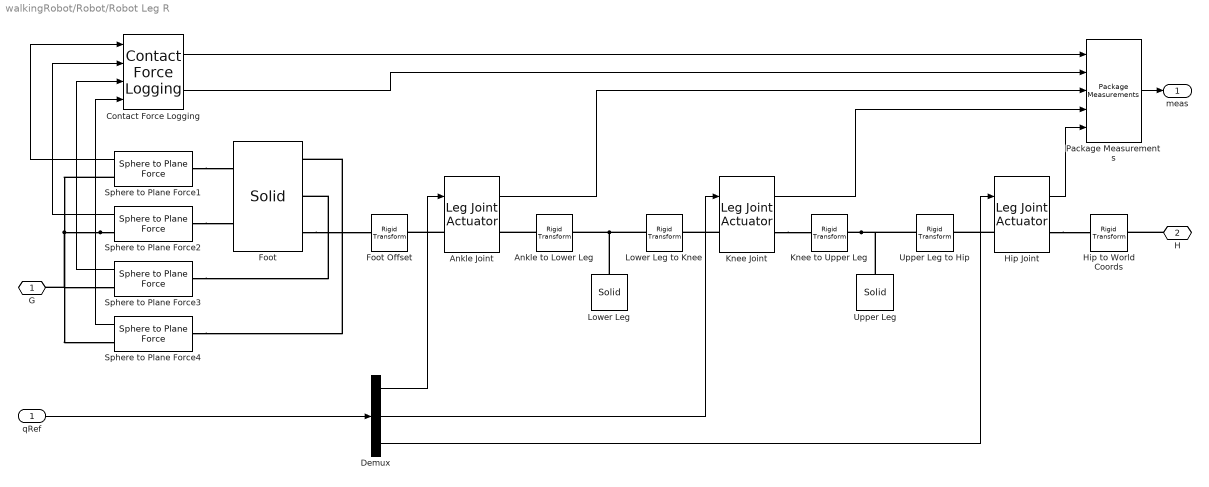
== system walkingRobot/Robot/Robot Leg R ==
  qRef : Inport
  Ankle Joint : walkingRobotUtils/Leg Joint Actuator  k=joint_stiffness  d=joint_damping  initAngle=initAnglesR(1)  Tf=motion_time_constant  Kp=ankle_servo_kp  Ki=ankle_servo_ki  Kd=ankle_servo_kd  N=deriv_filter_coeff  Tmax=max_torque
  Ankle to Lower Leg : sm_lib/Frames and Transforms/Rigid Transform  TranslationMethod=Cartesian  TranslationStandardOffset=0  TranslationLengthUnit=cm  TranslationStandardAxis=+Z  TranslationCartesianOffset=[0 lower_leg_length/2 0]  TranslationROffset=0  TranslationROffsetUnits=m  TranslationZOffset=0  TranslationZOffsetUnits=m  TranslationThetaOffset=0  TranslationThetaOffsetUnits=deg  RotationMethod=StandardAxis  RotationAngleUnits=deg  RotationStandardAxis=+X  RotationAngle=-90  RotationArbitraryAxis=[0 0 1]  FollAlignAxisA=+X  BaseAlignAxisA=+Y  FollAlignAxisB=+Y  BaseAlignAxisB=+Z  RotationSequenceAxes=FollowerAxes  RotationSequence=XYX  RotationSequenceAngles=[0 0 0]  RotationSequenceAnglesUnits=deg  RotationMatrix=[1 0 0; 0 1 0; 0 0 1]
  Contact Force Logging : walkingRobotUtils/Contact Force Logging  SystemSampleTime=-1
  Demux : Demux  Outputs=3
  Foot : sm_lib/Body Elements/Solid  InertiaType=CalculateFromGeometry  Mass=1  MassUnits=kg  CenterOfMass=[0 0 0]  CenterOfMassUnits=m  MomentsOfInertia=[1 1 1]  MomentsOfInertiaUnits=kg*m^2  ProductsOfInertia=[0 0 0]  ProductsOfInertiaUnits=kg*m^2  BasedOnType=Density  Density=foot_density  DensityUnits=kg/(m^3)  DoExposeReferenceFrame=off  SerializedFrames=<Frames><Frame><Id>Frame1</Id><Value><Name>F1</Name><Origin><Source>GeometricFeature</Source><FeatureName>+x -y -z point</FeatureName></Origin><PrimaryAxis><DefinedDirection>+Z</DefinedDirection><Source>ReferenceFrame</Source><SourceDirection>+Z</SourceDirection><FeatureName></FeatureName></PrimaryAxis><SecondaryAxis><DefinedDirection>+X</DefinedDirection><Source>ReferenceFrame</Source><SourceDirection>+X</SourceDirection><FeatureName></FeatureName></SecondaryAxis></Value></Frame><Frame><Id>Frame2</Id><Value><Name>F2</Name><Origin><Source>GeometricFeature</Source><FeatureName>+x +y -z point</FeatureName></Origin><PrimaryAxis><DefinedDirection>+Z</DefinedDirection><Source>ReferenceFrame</Source><SourceDirection>+Z</SourceDirection><FeatureName></FeatureName></PrimaryAxis><SecondaryAxis><DefinedDirection>+X</DefinedDirection><Source>ReferenceFrame</Source><SourceDirection>+X</SourceDirection><FeatureName></FeatureName></SecondaryAxis></Value></Frame><Frame><Id>Frame3</Id><Value><Name>F3</Name><Origin><Source>GeometricFeature</Source><FeatureName>-x -y -z point</FeatureName></Origin><PrimaryAxis><DefinedDirection>+Z</DefinedDirection><Source>ReferenceFrame</Source><SourceDirection>+Z</SourceDirection><FeatureName></FeatureName></PrimaryAxis><SecondaryAxis><DefinedDirection>+X</DefinedDirection><Source>ReferenceFrame</Source><SourceDirection>+X</SourceDirection><FeatureName></FeatureName></SecondaryAxis></Value></Frame><Frame><Id>Frame4</Id><Value><Name>F4</Name><Origin><Source>GeometricFeature</Source><FeatureName>-x +y -z point</FeatureName></Origin><PrimaryAxis><DefinedDirection>+Z</DefinedDirection><Source>ReferenceFrame</Source><SourceDirection>+Z</SourceDirection><FeatureName></FeatureName></PrimaryAxis><SecondaryAxis><DefinedDirection>+X</DefinedDirection><Source>ReferenceFrame</Source><SourceDirection>+X</SourceDirection><FeatureName></FeatureName></SecondaryAxis></Value></Frame><Frame><Id>Frame5</Id><Value><Name>A</Name><Origin><Source>GeometricFeature</Source><FeatureName>+z surface</FeatureName></Origin><PrimaryAxis><DefinedDirection>+Z</DefinedDirection><Source>ReferenceFrame</Source><SourceDirection>-Y</SourceDirection><FeatureName></FeatureName></PrimaryAxis><SecondaryAxis><DefinedDirection>+X</DefinedDirection><Source>ReferenceFrame</Source><SourceDirection>+X</SourceDirection><FeatureName></FeatureName></SecondaryAxis></Value></Frame></Frames>  GraphicType=FromGeometry  MarkerShape=Sphere  MarkerSize=10  MarkerSizeUnits=m  GraphicVisPropType=SimpleVisualProperties  GraphicDiffuseColor=[0.5 0.5 0.5]  GraphicSpecularColor=[0.5 0.5 0.5 1.0]  GraphicAmbientColor=[0.15 0.15 0.15 1.0]  GraphicEmissiveColor=[0.0 0.0 0.0 1.0]  GraphicShininess=75  GraphicOpacity=1.0  GeometryShape=Brick  RectangleSize=[1 1]  RectangleSizeUnits=m  BrickDimensions=[foot_x foot_y foot_z]  BrickDimensionUnits=cm  CylinderRadius=1  CylinderRadiusUnits=m  CylinderLength=1  CylinderLengthUnits=m  SphereRadius=1  SphereRadiusUnits=m  EllipsoidRadii=[1 1 1]  EllipsoidRadiiUnits=m  ExtrusionCrossSection=[1 1; -1 1; -1 -1; 1 -1]  ExtrusionCrossSectionUnits=m  ExtrusionLength=1  ExtrusionLengthUnits=m  PolygonNumSides=3  PolygonOuterRadius=1  PolygonOuterRadiusUnits=m  ExtGeomFileType=STL  ExtGeomFileUnits=m  RevolutionCrossSection=[1 1; 1 -1; 2 -1; 2 1]  RevolutionCrossSectionUnits=m  RevolutionExtent=Full  RevolutionAngle=180  RevolutionAngleUnits=deg
  Foot Offset : sm_lib/Frames and Transforms/Rigid Transform  TranslationMethod=Cartesian  TranslationStandardOffset=0  TranslationLengthUnit=cm  TranslationStandardAxis=+Z  TranslationCartesianOffset=foot_offset  TranslationROffset=0  TranslationROffsetUnits=m  TranslationZOffset=0  TranslationZOffsetUnits=m  TranslationThetaOffset=0  TranslationThetaOffsetUnits=deg  RotationMethod=None  RotationAngleUnits=deg  RotationStandardAxis=+X  RotationAngle=-90  RotationArbitraryAxis=[0 0 1]  FollAlignAxisA=+X  BaseAlignAxisA=+Y  FollAlignAxisB=+Y  BaseAlignAxisB=+Z  RotationSequenceAxes=FollowerAxes  RotationSequence=XYX  RotationSequenceAngles=[0 0 0]  RotationSequenceAnglesUnits=deg  RotationMatrix=[1 0 0; 0 1 0; 0 0 1]
  Hip Joint : walkingRobotUtils/Leg Joint Actuator  k=joint_stiffness  d=joint_damping  initAngle=initAnglesR(3)  Tf=motion_time_constant  Kp=hip_servo_kp  Ki=hip_servo_ki  Kd=hip_servo_kd  N=deriv_filter_coeff  Tmax=max_torque
  Hip to World Coords : sm_lib/Frames and Transforms/Rigid Transform  TranslationMethod=None  TranslationStandardOffset=0  TranslationLengthUnit=cm  TranslationStandardAxis=+Z  TranslationCartesianOffset=[0 0 upper_leg_length/2]  TranslationROffset=0  TranslationROffsetUnits=m  TranslationZOffset=0  TranslationZOffsetUnits=m  TranslationThetaOffset=0  TranslationThetaOffsetUnits=deg  RotationMethod=StandardAxis  RotationAngleUnits=deg  RotationStandardAxis=+X  RotationAngle=-90  RotationArbitraryAxis=[0 0 1]  FollAlignAxisA=+X  BaseAlignAxisA=+Y  FollAlignAxisB=+Y  BaseAlignAxisB=+Z  RotationSequenceAxes=FollowerAxes  RotationSequence=XYX  RotationSequenceAngles=[0 0 0]  RotationSequenceAnglesUnits=deg  RotationMatrix=[1 0 0; 0 1 0; 0 0 1]
  Knee Joint : walkingRobotUtils/Leg Joint Actuator  k=joint_stiffness  d=joint_damping  initAngle=initAnglesR(2)  Tf=motion_time_constant  Kp=knee_servo_kp  Ki=knee_servo_ki  Kd=knee_servo_kd  N=deriv_filter_coeff  Tmax=max_torque
  Knee to Upper Leg : sm_lib/Frames and Transforms/Rigid Transform  TranslationMethod=Cartesian  TranslationStandardOffset=0  TranslationLengthUnit=cm  TranslationStandardAxis=+Z  TranslationCartesianOffset=[0 upper_leg_length/2 0]  TranslationROffset=0  TranslationROffsetUnits=m  TranslationZOffset=0  TranslationZOffsetUnits=m  TranslationThetaOffset=0  TranslationThetaOffsetUnits=deg  RotationMethod=StandardAxis  RotationAngleUnits=deg  RotationStandardAxis=+X  RotationAngle=-90  RotationArbitraryAxis=[0 0 1]  FollAlignAxisA=+X  BaseAlignAxisA=+Y  FollAlignAxisB=+Y  BaseAlignAxisB=+Z  RotationSequenceAxes=FollowerAxes  RotationSequence=XYX  RotationSequenceAngles=[0 0 0]  RotationSequenceAnglesUnits=deg  RotationMatrix=[1 0 0; 0 1 0; 0 0 1]
  Lower Leg : sm_lib/Body Elements/Solid  InertiaType=CalculateFromGeometry  Mass=1  MassUnits=kg  CenterOfMass=[0 0 0]  CenterOfMassUnits=m  MomentsOfInertia=[1 1 1]  MomentsOfInertiaUnits=kg*m^2  ProductsOfInertia=[1 1 1]  ProductsOfInertiaUnits=kg*m^2  BasedOnType=Density  Density=density  DensityUnits=kg/m^3  DoExposeReferenceFrame=on  SerializedFrames=<Frames/>  GraphicType=FromGeometry  MarkerShape=Sphere  MarkerSize=10  GraphicVisPropType=SimpleVisualProperties  GraphicDiffuseColor=[0.4 0.4 1.0]  GraphicSpecularColor=[0.5 0.5 0.5 1.0]  GraphicAmbientColor=[0.15 0.15 0.15 1.0]  GraphicEmissiveColor=[0.0 0.0 0.0 1.0]  GraphicShininess=75  GraphicOpacity=1.0  GeometryShape=Cylinder  RectangleSize=[1 1]  RectangleSizeUnits=m  BrickDimensions=[1 1 1]  BrickDimensionUnits=m  CylinderRadius=leg_radius  CylinderRadiusUnits=cm  CylinderLength=lower_leg_length  CylinderLengthUnits=cm  SphereRadius=1  SphereRadiusUnits=m  EllipsoidRadii=[1 1 1]  EllipsoidRadiiUnits=m  ExtrusionCrossSection=[1 1; -1 1; -1 -1; 1 -1]  ExtrusionCrossSectionUnits=m  ExtrusionLength=1  ExtrusionLengthUnits=m  PolygonNumSides=3  PolygonOuterRadius=1  PolygonOuterRadiusUnits=m  ExtGeomFileType=STEP  ExtGeomFileUnits=m  RevolutionCrossSection=[1 1; 1 -1; 2 -1; 2 1]  RevolutionCrossSectionUnits=m  RevolutionExtent=Full  RevolutionAngle=180  RevolutionAngleUnits=deg
  Lower Leg to Knee : sm_lib/Frames and Transforms/Rigid Transform  TranslationMethod=Cartesian  TranslationStandardOffset=0  TranslationLengthUnit=cm  TranslationStandardAxis=+Z  TranslationCartesianOffset=[0 0 lower_leg_length/2]  TranslationROffset=0  TranslationROffsetUnits=m  TranslationZOffset=0  TranslationZOffsetUnits=m  TranslationThetaOffset=0  TranslationThetaOffsetUnits=deg  RotationMethod=StandardAxis  RotationAngleUnits=deg  RotationStandardAxis=+X  RotationAngle=90  RotationArbitraryAxis=[0 0 1]  FollAlignAxisA=+X  BaseAlignAxisA=+Y  FollAlignAxisB=+Y  BaseAlignAxisB=+Z  RotationSequenceAxes=FollowerAxes  RotationSequence=XYX  RotationSequenceAngles=[0 0 0]  RotationSequenceAnglesUnits=deg  RotationMatrix=[1 0 0; 0 1 0; 0 0 1]
  Package Measurements : walkingRobotUtils/Package  Measurements  SystemSampleTime=-1
  Sphere to Plane Force{1..4} (4 alike) : Contact_Forces_Lib/3D/Sphere to Plane Force  sphere_rad=contact_point_radius  plane_lenx=plane_x  plane_leny=plane_y  plane_depth=height_plane/2  force_law=Linear  k_contact=contact_stiffness  b_contact=contact_damping  pen_full_damp_F=1e-4  pen_exponent=1  custom_param_1=1  custom_param_2=1  friction_law=Stick-Slip Continuous  mu_kinetic=mu_k  mu_static=mu_s  v_thr=mu_vth  vis_on=off  vis_opc_en=0  vis_len_plaBz=0.005  vis_clr=[0.9 0.2 0.2]  vis_opc=0.7
  Upper Leg : sm_lib/Body Elements/Solid  InertiaType=CalculateFromGeometry  Mass=1  MassUnits=kg  CenterOfMass=[0 0 0]  CenterOfMassUnits=m  MomentsOfInertia=[1 1 1]  MomentsOfInertiaUnits=kg*m^2  ProductsOfInertia=[1 1 1]  ProductsOfInertiaUnits=kg*m^2  BasedOnType=Density  Density=density  DensityUnits=kg/m^3  DoExposeReferenceFrame=on  SerializedFrames=<Frames/>  GraphicType=FromGeometry  MarkerShape=Sphere  MarkerSize=10  GraphicVisPropType=SimpleVisualProperties  GraphicDiffuseColor=[1.0 0.4 0.4]  GraphicSpecularColor=[0.5 0.5 0.5 1.0]  GraphicAmbientColor=[0.15 0.15 0.15 1.0]  GraphicEmissiveColor=[0.0 0.0 0.0 1.0]  GraphicShininess=75  GraphicOpacity=1.0  GeometryShape=Cylinder  RectangleSize=[1 1]  RectangleSizeUnits=m  BrickDimensions=[1 1 1]  BrickDimensionUnits=m  CylinderRadius=leg_radius  CylinderRadiusUnits=cm  CylinderLength=upper_leg_length  CylinderLengthUnits=cm  SphereRadius=1  SphereRadiusUnits=m  EllipsoidRadii=[1 1 1]  EllipsoidRadiiUnits=m  ExtrusionCrossSection=[1 1; -1 1; -1 -1; 1 -1]  ExtrusionCrossSectionUnits=m  ExtrusionLength=1  ExtrusionLengthUnits=m  PolygonNumSides=3  PolygonOuterRadius=1  PolygonOuterRadiusUnits=m  ExtGeomFileType=STEP  ExtGeomFileUnits=m  RevolutionCrossSection=[1 1; 1 -1; 2 -1; 2 1]  RevolutionCrossSectionUnits=m  RevolutionExtent=Full  RevolutionAngle=180  RevolutionAngleUnits=deg
  Upper Leg to Hip : sm_lib/Frames and Transforms/Rigid Transform  TranslationMethod=Cartesian  TranslationStandardOffset=0  TranslationLengthUnit=cm  TranslationStandardAxis=+Z  TranslationCartesianOffset=[0 0 upper_leg_length/2]  TranslationROffset=0  TranslationROffsetUnits=m  TranslationZOffset=0  TranslationZOffsetUnits=m  TranslationThetaOffset=0  TranslationThetaOffsetUnits=deg  RotationMethod=StandardAxis  RotationAngleUnits=deg  RotationStandardAxis=+X  RotationAngle=90  RotationArbitraryAxis=[0 0 1]  FollAlignAxisA=+X  BaseAlignAxisA=+Y  FollAlignAxisB=+Y  BaseAlignAxisB=+Z  RotationSequenceAxes=FollowerAxes  RotationSequence=XYX  RotationSequenceAngles=[0 0 0]  RotationSequenceAnglesUnits=deg  RotationMatrix=[1 0 0; 0 1 0; 0 0 1]
  G : PMIOPort  Side=Right
  H : PMIOPort  Port=2  Side=Right
  meas : Outport
  wires:
  qRef/1 -> Demux/1
  Sphere to Plane Force4/1 -> Contact Force Logging/4
  Sphere to Plane Force3/1 -> Contact Force Logging/3
  Sphere to Plane Force2/1 -> Contact Force Logging/2
  Sphere to Plane Force1/1 -> Contact Force Logging/1
  Ankle Joint/1 -> Package Measurements/3
  Knee Joint/1 -> Package Measurements/4
  Hip Joint/1 -> Package Measurements/5
  Package Measurements/1 -> meas/1
  Demux/3 -> Hip Joint/1
  Demux/2 -> Knee Joint/1
  Demux/1 -> Ankle Joint/1
  Contact Force Logging/2 -> Package Measurements/2
  Contact Force Logging/1 -> Package Measurements/1
  connections:
  Foot/LConn3 -- Foot Offset/LConn1
  Hip Joint/RConn1 -- Hip to World Coords/LConn1
  H/RConn1 -- Hip to World Coords/RConn1
  Knee Joint/LConn1 -- Lower Leg to Knee/RConn1
  Hip Joint/LConn1 -- Upper Leg to Hip/RConn1
  Knee to Upper Leg/RConn1 -- Upper Leg/RConn1 -- Upper Leg to Hip/LConn1
  Ankle Joint/LConn1 -- Foot Offset/RConn1
  Lower Leg to Knee/LConn1 -- Lower Leg/RConn1 -- Ankle to Lower Leg/RConn1
  Sphere to Plane Force3/LConn1 -- Foot/LConn2
  Sphere to Plane Force4/LConn1 -- Foot/LConn1
  Sphere to Plane Force1/LConn1 -- Foot/RConn1
  Sphere to Plane Force2/LConn1 -- Foot/RConn2
  Ankle to Lower Leg/LConn1 -- Ankle Joint/RConn1
  Knee Joint/RConn1 -- Knee to Upper Leg/LConn1
  Sphere to Plane Force2/RConn1 -- Sphere to Plane Force1/RConn1 -- Sphere to Plane Force3/RConn1 -- Sphere to Plane Force4/RConn1 -- G/RConn1
